simulink model "testing"  (R2025a)
settings: Solver=VariableStepAuto  StartTime=0.0  StopTime=10  RelTol=1e-3
model workspace (MAT data in the model file):
  Kphi = 3
  Ks = 1
  Ky = 0.5
  L = 2.7
  Sig = Simulink.Signal
  Sig.Dimensions = -1
  Sig.DimensionsMode = 'auto'
  Sig.Complexity = 'auto'
  Sig.SampleTime = -1
  Sig.SamplingMode = 'auto'
  Sig.DataType = 'auto'
  delta0 = 0
  delta_max = 0.5
  ephi0 = 0
  ey0 = 1
  tau_s = 0.1
  v = 30
settings Model: Creator=GIGABYTE  LastModifiedBy=GIGABYTE

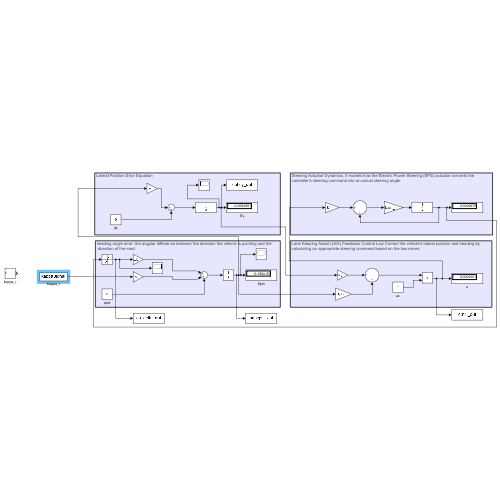
[thumbnail: Simulink's stored preview of the top-level diagram]
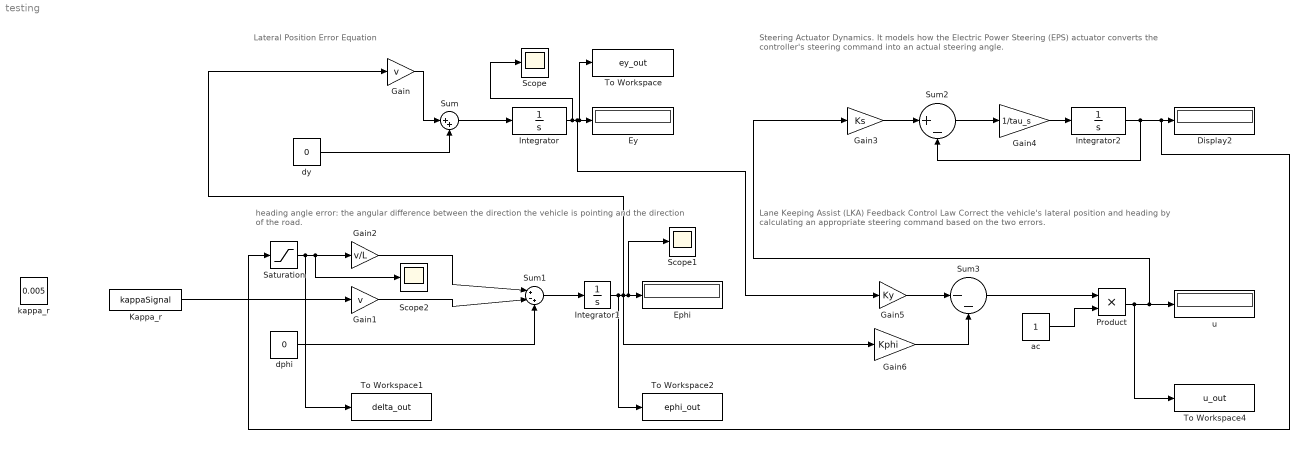
== system testing ==
  note: Lane Keeping Assist (LKA) Feedback Control Law Correct the vehicle's lateral position and heading by
      | calculating an appropriate steering command based on the two errors.
  note: Steering Actuator Dynamics. It models how the Electric Power Steering (EPS) actuator converts the
      | controller's steering command into an actual steering angle.
  note: heading angle error: the angular difference between the direction the vehicle is pointing and the
      |  direction of the road.
  note: Lateral Position Error Equation
  Display2 : Display
  Ephi : Display
  Ey : Display
  Gain : Gain  Gain=v
  Gain1 : Gain  Gain=v
  Gain2 : Gain  Gain=v/L
  Gain3 : Gain  Gain=Ks
  Gain4 : Gain  Gain=1/tau_s
  Gain5 : Gain  Gain=Ky
  Gain6 : Gain  Gain=Kphi
  Integrator : Integrator  InitialCondition=ey0
  Integrator1 : Integrator  InitialCondition=ephi0
  Integrator2 : Integrator  InitialCondition=delta0
  Kappa_r : FromWorkspace  VariableName=kappaSignal
  Product : Product
  Saturation : Saturate
  Scope : Scope
      settings: ActiveDisplayYMinimum=-0.20086481627142219  ActiveDisplayYMaximum=1.1334294240301581
  Scope1 : Scope
      settings: ActiveDisplayYMinimum=-1  ActiveDisplayYMaximum=1
  Scope2 : Scope
      settings: ActiveDisplayYMinimum=-0.3607666101634614  ActiveDisplayYMaximum=0.37071060205861572  DataLoggingVariableName=ScopeData2
  Sum : Sum  Inputs=|++
  Sum1 : Sum  Inputs=|+-+
  Sum2 : Sum  Inputs=|+-
  Sum3 : Sum  Inputs=|--
  To Workspace : ToWorkspace  VariableName=ey_out  SaveFormat=Timeseries  SampleTime=-1
  To Workspace1 : ToWorkspace  VariableName=delta_out  SaveFormat=Timeseries  SampleTime=-1
  To Workspace2 : ToWorkspace  VariableName=ephi_out  SaveFormat=Timeseries  SampleTime=-1
  To Workspace4 : ToWorkspace  VariableName=u_out  SaveFormat=Timeseries  SampleTime=-1
  ac : Constant
  dphi : Constant  Value=0
  dy : Constant  Value=0
  kappa_r : Constant  Value=0.005
  u : Display
  wires:
  Gain/1 -> Sum/1
  Sum/1 -> Integrator/1
  Integrator/1 -> Scope/1, Gain5/1, To Workspace/1, Ey/1
  dy/1 -> Sum/2
  Gain2/1 -> Sum1/1
  Gain1/1 -> Sum1/2
  dphi/1 -> Sum1/3
  Sum1/1 -> Integrator1/1
  Integrator1/1 -> To Workspace2/1, Gain6/1, Gain/1, Scope1/1, Ephi/1
  Gain3/1 -> Sum2/1
  Sum2/1 -> Gain4/1
  Gain4/1 -> Integrator2/1
  Integrator2/1 -> Sum2/2, Saturation/1, Display2/1
  Gain5/1 -> Sum3/1
  Gain6/1 -> Sum3/2
  Saturation/1 -> To Workspace1/1, Scope2/1, Gain2/1
  Product/1 -> To Workspace4/1, Gain3/1, u/1
  Sum3/1 -> Product/1
  ac/1 -> Product/2
  Kappa_r/1 -> Gain1/1
